simulink model "r2_b16a4x512f"  (R2012b)
settings: Solver=VariableStepDiscrete  SolverMode=SingleTasking  StartTime=0.0  StopTime=1  RelTol=1e-3
undefined symbols (not defined in the file): fft_stages, n_bits_ants, n_bits_xengs
libraries: xbsIndex_r4 x27410, casper_library_misc x230, xbsReplacements_r4 x24, casper_library_delays x8, xps_library x5, casper_library_communications x4
(part 90 of 229)

== system r2_b16a4x512f/sys3/pkt_reord_devel/munge1 ==
  din : Inport
  join : Subsystem  AncestorBlock=casper_library_flow_control/bus_create  mask(bus_create){inputNum=2}
      mask prompts: inputNum "Number of inputs:"
      mask init:
      | bus_create_init(gcb,...
      |     'inputNum', inputNum);
  reinterpret : xbsIndex_r4/Reinterpret  force_arith_type=on  arith_type=Unsigned  force_bin_pt=on  bin_pt=0  block_type=reinterpret
  reinterpret_out : xbsIndex_r4/Reinterpret  force_arith_type=on  arith_type=Unsigned  force_bin_pt=on  bin_pt=0  block_type=reinterpret
  split : Subsystem  AncestorBlock=casper_library_flow_control/bus_expand  mask(bus_expand){mode=divisions of arbitrary size, outputNum=1, outputWidth=[1 32], outputBinaryPt=[0 0], outputArithmeticType=[0 0], show_format=off, outputToWorkspace=off, variablePrefix=out, outputToModelAsWell=on}
      mask prompts: outputNum "Number of outputs:"; outputWidth "Output width [msb ... lsb]:"; outputBinaryPt "Output binary point position [msb ... lsb]:"; outputArithmeticType "Output arithmetic type (ufix=0, fix=1, bool=2) [msb ... lsb]:"; show_format "Print format string?"; outputToWorkspace "Output to workspace?"; variablePrefix "Variable name prefix:"; outputToModelAsWell "Output to model as well?"
      mask help:
      | Expands a 'bus' made using a bus_create or Xilinx
      | concat block.
      | The input will be divided into the specified number
      | of outputs with the specified arithmetic types.
      | Divisions are made from most significant bit.
      mask init: same as r2_b16a4x512f/bus_expand
      settings: AttributesFormatString=2 outputs
      mask TypeOptions mode: divisions of equal size | divisions of arbitrary size
      mask Callback mode: bus_expand_callback();
      mask Callback outputWidth: bus_expand_callback();
      mask Callback outputToWorkspace: bus_expand_callback();
  dout : Outport
  wires:
  split/2(lsb_out1) -> join/2(in2)
  split/1(msb_out2) -> join/1(in1)
  join/1(bus_out) -> reinterpret_out/1
  reinterpret/1 -> split/1(bus_in)
  din/1 -> reinterpret/1
  reinterpret_out/1 -> dout/1

== system r2_b16a4x512f/sys3/pkt_reord_devel/output_control ==
  note: rd_addr is counting for
      | output words to
      | X engines
  note: If the read window is 1/2
      | the total buffer size (or more)
      | behind the write window,
      | it is time to ship it out.
  note: Decide whether to ship
      | a window or not:
  note: If we need to ship a window,
      | send the data on a window edge
  note: If reading from addr 0 (corresponding to f=0,nant,2nant,...)
      | and max_mcnt (skipping window_bits for the difference
      | between max_mcnt and rd_mcnt) is 0 for sync_bits, then
      | issue a sync.
  note: add delay here
      | to ensure mcnt has had
      | chance to calculate
      | correctly
  maxcnt : Inport
  AddSub1 : xbsIndex_r4/AddSub  mode=Subtraction  use_carryin=off  use_carryout=off  en=off  latency=2  precision=User Defined  arith_type=Unsigned  n_bits=window_bits  bin_pt=0  quantization=Truncate  overflow=Wrap  dbl_ovrd=off  use_behavioral_HDL=on  hw_selection=Fabric  pipelined=off  use_rpm=on  block_type=addsub
      settings: xl_area=[0, 0, 0, 0, 0, 0, 0]  block_version=10.1.3
  Concat1 : xbsIndex_r4/Concat  num_inputs=2  dbl_ovrd=off  block_type=concat
      settings: block_version=10.1.3
  Concat2 : xbsIndex_r4/Concat  num_inputs=2  dbl_ovrd=off  block_type=concat
      settings: block_version=10.1.3
  Constant1 : xbsIndex_r4/Constant  const=2^(window_bits - 1)  gui_display_data_type=Fixed-point  arith_type=Unsigned  n_bits=window_bits  bin_pt=0  preci_type=Single  exp_width=8  frac_width=24  explicit_period=on  period=1  equ=P=C  opselect=C  inp2=PCIN>>17  opr=+  inp1=P  carry=CIN  dbl_ovrd=off  block_type=constant
  Constant3 : xbsIndex_r4/Constant  const=0  gui_display_data_type=Fixed-point  arith_type=Unsigned  n_bits=sync_bits - x_int_bits - ant_bits - window_bits  bin_pt=0  preci_type=Single  exp_width=8  frac_width=24  explicit_period=on  period=1  equ=P=C  opselect=C  inp2=PCIN>>17  opr=+  inp1=P  carry=CIN  dbl_ovrd=off  block_type=constant
  Delay1 : xbsIndex_r4/Delay  rst=off  infoeditControl=Selection of Reset will increase slice count due to use of real FFs and instead of SRLs  en=off  latency=1  dbl_ovrd=off  reg_retiming=on  block_type=delay
      settings: xl_area=[0, 0, 0, 0, 0, 0, 0]
  Delay3 : xbsIndex_r4/Delay  rst=off  infoeditControl=Selection of Reset will increase slice count due to use of real FFs and instead of SRLs  en=off  latency=2  dbl_ovrd=off  reg_retiming=on  block_type=delay
      settings: xl_area=[0, 0, 0, 0, 0, 0, 0]
  Delay6 : xbsIndex_r4/Delay  rst=off  infoeditControl=Selection of Reset will increase slice count due to use of real FFs and instead of SRLs  en=off  latency=1  dbl_ovrd=off  reg_retiming=on  block_type=delay
      settings: xl_area=[0, 0, 0, 0, 0, 0, 0]
  Delay7 : xbsIndex_r4/Delay  rst=off  infoeditControl=Selection of Reset will increase slice count due to use of real FFs and instead of SRLs  en=off  latency=2  dbl_ovrd=off  reg_retiming=on  block_type=delay
      settings: xl_area=[0, 0, 0, 0, 0, 0, 0]
  Gateway Out{1..18} (18 alike) : xbsIndex_r4/Gateway Out  inherit_from_input=off  hdl_port=off  timing_constraint=None  locs_specified=off  LOCs={}  UseAsDAC=off  DACChannel='1'  block_type=gatewayout
      settings: infoedit="Gateway out block.  Converts Xilinx fixed point inputs into ouputs of type Simulink integer, double, or fixed point.<P><P>Hardware notes:  In hardware these blocks become top level output ports or are discarded, depending on how they are configured."  xl_area=[0, 0, 0, 0, 0, 0, 0]  block_version=10.1.3
  Logical1 : xbsIndex_r4/Logical  logical_function=AND  inputs=2  en=off  latency=0  precision=Full  arith_type=Unsigned  n_bits=8  bin_pt=2  align_bp=on  dbl_ovrd=off  block_type=logical
      settings: xl_area=[0, 0, 0, 0, 0, 0, 0]
  Logical2 : xbsIndex_r4/Logical  logical_function=AND  inputs=2  en=off  latency=0  precision=Full  arith_type=Unsigned  n_bits=8  bin_pt=2  align_bp=on  dbl_ovrd=off  block_type=logical
      settings: xl_area=[0, 0, 0, 0, 0, 0, 0]
  Logical4 : xbsIndex_r4/Logical  logical_function=AND  inputs=2  en=off  latency=0  precision=Full  arith_type=Unsigned  n_bits=8  bin_pt=2  align_bp=on  dbl_ovrd=off  block_type=logical
      settings: xl_area=[0, 0, 0, 0, 0, 0, 0]
  Register : xbsIndex_r4/Register  init=0  rst=off  en=on  dbl_ovrd=off  block_type=register
  Register1 : xbsIndex_r4/Register  init=0  rst=off  en=on  dbl_ovrd=off  block_type=register
  Register3 : xbsIndex_r4/Register  init=0  rst=off  en=on  dbl_ovrd=off  block_type=register
  Relational1 : xbsIndex_r4/Relational  mode=a>=b  en=off  latency=1  dbl_ovrd=off  block_type=relational
      settings: xl_area=[0, 0, 0, 0, 0, 0, 0]  block_version=10.1.3
  Relational4 : xbsIndex_r4/Relational  mode=a=b  en=off  latency=1  dbl_ovrd=off  block_type=relational
      settings: xl_area=[0, 0, 0, 0, 0, 0, 0]  block_version=10.1.3
  Slice1 : xbsIndex_r4/Slice  nbits=window_bits  boolean_output=off  mode=Lower Bit Location + Width  bit1=0  base1=MSB of Input  bit0=0  base0=LSB of Input  dbl_ovrd=off  block_type=slice
      settings: infoedit="Extracts a given range of bits from each input sample and presents it at the output.  The output type is ordinarily unsigned with binary point at zero, but can be Boolean when the slice is one bit wide.<P><P>Hardware notes: In hardware this block costs nothing."  block_version=10.1.3
  Slice2 : xbsIndex_r4/Slice  nbits=1  boolean_output=on  mode=Upper Bit Location + Width  bit1=0  base1=MSB of Input  bit0=0  base0=LSB of Input  dbl_ovrd=off  block_type=slice
      settings: infoedit="Extracts a given range of bits from each input sample and presents it at the output.  The output type is ordinarily unsigned with binary point at zero, but can be Boolean when the slice is one bit wide.<P><P>Hardware notes: In hardware this block costs nothing."  block_version=10.1.3
  Slice3 : xbsIndex_r4/Slice  nbits=window_bits  boolean_output=off  mode=Lower Bit Location + Width  bit1=0  base1=MSB of Input  bit0=0  base0=LSB of Input  dbl_ovrd=off  block_type=slice
      settings: infoedit="Extracts a given range of bits from each input sample and presents it at the output.  The output type is ordinarily unsigned with binary point at zero, but can be Boolean when the slice is one bit wide.<P><P>Hardware notes: In hardware this block costs nothing."  block_version=10.1.3
  Slice4 : xbsIndex_r4/Slice  nbits=x_int_bits + ant_bits - n_bits_output_words  boolean_output=off  mode=Lower Bit Location + Width  bit1=0  base1=MSB of Input  bit0=0  base0=LSB of Input  dbl_ovrd=off  block_type=slice
      settings: block_version=10.1.3
  Slice5 : xbsIndex_r4/Slice  nbits=window_bits  boolean_output=off  mode=Two Bit Locations  bit1=sync_bits - x_int_bits - ant_bits - 1  base1=LSB of Input  bit0=window_bits  base0=LSB of Input  dbl_ovrd=off  block_type=slice
      settings: infoedit="Extracts a given range of bits from each input sample and presents it at the output.  The output type is ordinarily unsigned with binary point at zero, but can be Boolean when the slice is one bit wide.<P><P>Hardware notes: In hardware this block costs nothing."  block_version=10.1.3
  Slice6 : xbsIndex_r4/Slice  nbits=1  boolean_output=on  mode=Upper Bit Location + Width  bit1=0  base1=MSB of Input  bit0=0  base0=LSB of Input  dbl_ovrd=off  block_type=slice
      settings: infoedit="Extracts a given range of bits from each input sample and presents it at the output.  The output type is ordinarily unsigned with binary point at zero, but can be Boolean when the slice is one bit wide.<P><P>Hardware notes: In hardware this block costs nothing."  block_version=10.1.3
  Slice7 : xbsIndex_r4/Slice  nbits=1  boolean_output=off  mode=Two Bit Locations  bit1=0  base1=MSB of Input  bit0=window_bits  base0=LSB of Input  dbl_ovrd=off  block_type=slice
      settings: infoedit="Extracts a given range of bits from each input sample and presents it at the output.  The output type is ordinarily unsigned with binary point at zero, but can be Boolean when the slice is one bit wide.<P><P>Hardware notes: In hardware this block costs nothing."  block_version=10.1.3
  edge_detect : Subsystem  AncestorBlock=casper_library_misc/edge_detect  mask(edge_detect){edge=Both, polarity=Active High, x_in=[0 0.08 0.08 0.16 0.16 0.24 0.24 0.32 0.32 0.4], y_in=[-1 -1  1  1  1  1  1  1  1  1], x_out=[0.6 0.68 0.68 0.76 0.76 0.84 0.84 0.92 0.92 1], y_out=[-1 -1  1  1 -1 -1 -1 -1 -1 -1]}
      mask prompts: edge "Edge Type"; polarity "Output Polarity"; x_in "Input X Positions"; y_in "Input Y Positions"; x_out "Output X Positions"; y_out "Output Y Positions"
      mask help: Output is active for one-cycle after each edge of the specified type (i.e. rising, falling or both).
      mask init: same as r2_b16a4x512f/edge_detect
      settings: AttributesFormatString=|
      | both edges
      | active high
      mask Help: Output is active for one-cycle after each edge of the specified type (i.e. rising, falling, or both).  Latency is zero.
      mask TypeOptions edge: Rising | Falling | Both
      mask TypeOptions polarity: Active High | Active Low
      mask Display:
      | plot(x_in_num,0.5+y_in_num*0.2);
      | plot(x_out_num,0.5+y_out_num*0.2);
  edge_detect1 : Subsystem  AncestorBlock=casper_library_misc/edge_detect  mask(edge_detect){edge=Both, polarity=Active High, x_in=[0 0.08 0.08 0.16 0.16 0.24 0.24 0.32 0.32 0.4], y_in=[-1 -1  1  1  1  1  1  1  1  1], x_out=[0.6 0.68 0.68 0.76 0.76 0.84 0.84 0.92 0.92 1], y_out=[-1 -1  1  1 -1 -1 -1 -1 -1 -1]}
      mask prompts: edge "Edge Type"; polarity "Output Polarity"; x_in "Input X Positions"; y_in "Input Y Positions"; x_out "Output X Positions"; y_out "Output Y Positions"
      mask help: Output is active for one-cycle after each edge of the specified type (i.e. rising, falling or both).
      mask init: same as r2_b16a4x512f/edge_detect
      settings: AttributesFormatString=|
      | both edges
      | active high
      mask Help: Output is active for one-cycle after each edge of the specified type (i.e. rising, falling, or both).  Latency is zero.
      mask TypeOptions edge: Rising | Falling | Both
      mask TypeOptions polarity: Active High | Active Low
      mask Display:
      | plot(x_in_num,0.5+y_in_num*0.2);
      | plot(x_out_num,0.5+y_out_num*0.2);
  internal_descr_Scope : Scope  NumInputPorts=8
      settings: TimeRange=1  YMin=-1~-1~0.95~-5~-5~-5~-5~-5  YMax=1~1~1.05~5~5~5~5~5  SaveName=ScopeData2
  internal_descr_Scope1 : Scope  NumInputPorts=10
      settings: TimeRange=42.38350921521942  YMin=100.7~0~0~0~402.8~0.95~304~-1~-5~-5  YMax=111.3~10~80~1024~445.2~1.05~336~1~5~5  SaveName=ScopeData4
  pulse_ext : Subsystem  AncestorBlock=casper_library/Misc/pulse_ext  mask(pulse_ext){pulse_len=2^(x_int_bits + ant_bits)}
      mask prompts: pulse_len "Length of Pulse"
      mask help:
      | Extends a boolean signal to be high for the specified number of clocks after
      | the last high input.
      mask init:
      | bits = ceil(log2(pulse_len+1));
      mask Help: eval('xlWeb([getenv(''MLIB_ROOT''), ''\doc\htmlblocks\sp_pulse_ext\sp_pulse_ext.html''])')
  win_addr_cnt : xbsIndex_r4/Counter  cnt_type=Free Running  cnt_to=Inf  operation=Up  start_count=0  cnt_by_val=1  arith_type=Unsigned  n_bits=x_int_bits + ant_bits + 1 - n_bits_output_words  bin_pt=0  load_pin=off  rst=off  en=off  explicit_period=on  period=1  dbl_ovrd=off  use_behavioral_HDL=off  implementation=Fabric  use_rpm=on  block_type=counter
      settings: xl_area=[0, 0, 0, 0, 0, 0, 0]
  win_cnt : xbsIndex_r4/Counter  cnt_type=Free Running  cnt_to=Inf  operation=Up  start_count=0  cnt_by_val=1  arith_type=Unsigned  n_bits=window_bits + 1  bin_pt=0  load_pin=off  rst=off  en=on  explicit_period=off  period=1  dbl_ovrd=off  use_behavioral_HDL=off  implementation=Fabric  use_rpm=on  block_type=counter
      settings: xl_area=[0, 0, 0, 0, 0, 0, 0]
  gen_sync : Outport
  rd_en : Outport  Port=2
  rd_addr : Outport  Port=3
  rd_timefreq : Outport  Port=4
  wires:
  Concat2/1 -> [rd_mcnt], rd_timefreq/1
  Concat1/1 -> rd_addr/1, [rd_addr]
  Delay7/1 -> Concat1/2
  Slice2/1 -> edge_detect/1(in)
  Slice1/1 -> [current_window], Delay1/1
  Slice4/1 -> Delay7/1
  edge_detect1/1(out) -> Logical1/1
  Slice6/1 -> edge_detect1/1(in)
  win_addr_cnt/1 -> Slice4/1, Slice6/1
  Slice5/1 -> Relational4/2
  Constant3/1 -> Relational4/1
  edge_detect/1(out) -> Logical2/1, [buffer_edge]
  Logical1/1 -> Register3/1, Register3/2, pulse_ext/1(in), [ship_window_now]
  Register1/1 -> Slice2/1, Slice1/1
  maxcnt/1 -> Slice5/1, [maxcnt]
  [ship_next_window] -> Delay3/1
  Slice3/1 -> AddSub1/1
  AddSub1/1 -> Relational1/1
  Constant1/1 -> Relational1/2
  [current_window] -> AddSub1/2
  [maxcnt] -> Slice3/1
  Relational1/1 -> [ship_next_window]
  [ship_window_now] -> win_cnt/1, Register1/2
  Relational4/1 -> Logical2/2
  Gateway Out3/1 -> internal_descr_Scope/2
  Gateway Out4/1 -> internal_descr_Scope/1
  Gateway Out5/1 -> internal_descr_Scope/3
  [maxcnt] -> Gateway Out4/1
  [current_window_out] -> Gateway Out3/1
  [ship_next_window] -> Gateway Out5/1
  Gateway Out6/1 -> internal_descr_Scope/4
  Gateway Out1/1 -> internal_descr_Scope/5
  Gateway Out2/1 -> internal_descr_Scope/6
  [ship_window_now] -> Gateway Out6/1
  Gateway Out7/1 -> internal_descr_Scope/7
  [current_window_out] -> Concat2/2
  Gateway Out10/1 -> internal_descr_Scope1/2
  Gateway Out11/1 -> internal_descr_Scope1/1
  Gateway Out12/1 -> internal_descr_Scope1/3
  Gateway Out13/1 -> internal_descr_Scope1/4
  Gateway Out8/1 -> internal_descr_Scope1/5
  Gateway Out9/1 -> internal_descr_Scope1/6
  Gateway Out14/1 -> internal_descr_Scope1/7
  Gateway Out15/1 -> internal_descr_Scope1/8
  [gen_sync] -> Gateway Out15/1
  [gen_sync] -> Gateway Out16/1
  Gateway Out16/1 -> internal_descr_Scope/8
  Logical2/1 -> gen_sync/1, [gen_sync]
  [rd_mcnt] -> Gateway Out7/1
  Logical4/1 -> rd_en/1, [rd_en]
  pulse_ext/1(out) -> Delay6/1
  Register3/1 -> Logical4/2
  Delay6/1 -> Logical4/1
  win_cnt/1 -> Register1/1
  Delay1/1 -> [current_window_out]
  [current_window_out] -> Gateway Out11/1
  [maxcnt] -> Gateway Out10/1
  [offset_mcnt] -> Gateway Out12/1
  [ship_next_window] -> Gateway Out8/1
  [rd_mcnt] -> Gateway Out13/1
  [rd_en] -> Gateway Out9/1
  [rd_addr] -> Gateway Out14/1
  [rd_en] -> Gateway Out1/1
  [rd_addr] -> Gateway Out2/1
  [mcnt_sample] -> Gateway Out17/1
  Gateway Out17/1 -> internal_descr_Scope1/9
  Delay3/1 -> Logical1/2
  [maxcnt] -> Slice7/1, [offset_mcnt]
  Slice7/1 -> Register/1
  Register/1 -> Concat2/1, [sampled_mcnt]
  [sampled_mcnt] -> Gateway Out18/1
  Gateway Out18/1 -> internal_descr_Scope1/10
  [buffer_edge] -> Register/2, [mcnt_sample]
  [current_window_out] -> Concat1/1

== system r2_b16a4x512f/sys3/pkt_reord_devel/time_freq_unpack ==
  din : Inport
  xeng_id : Inport  Port=2
  Concat2 : xbsIndex_r4/Concat  num_inputs=2  dbl_ovrd=off  block_type=concat
  Slice2 : xbsIndex_r4/Slice  nbits=chan_bits-xeng_bits  boolean_output=off  mode=Lower Bit Location + Width  bit1=-1  base1=MSB of Input  bit0=0  base0=LSB of Input  dbl_ovrd=off  block_type=slice
      settings: block_version=10.1.3
  Slice3 : xbsIndex_r4/Slice  nbits=1  boolean_output=off  mode=Two Bit Locations  bit1=0  base1=MSB of Input  bit0=chan_bits-xeng_bits  base0=LSB of Input  dbl_ovrd=off  block_type=slice
      settings: block_version=10.1.3
  time : Outport
  freq : Outport  Port=2
  wires:
  din/1 -> Slice3/1, Slice2/1
  Slice3/1 -> time/1
  Slice2/1 -> Concat2/2
  Concat2/1 -> freq/1
  xeng_id/1 -> Concat2/1

== system r2_b16a4x512f/sys3/pre_process/bus_expand ==
  bus_in : Inport
  reinterpret{1..4} (4 alike) : xbsIndex_r4/Reinterpret  force_arith_type=on  arith_type=Unsigned  force_bin_pt=on  bin_pt=0  block_type=reinterpret
  slice1 : xbsIndex_r4/Slice  nbits=8  boolean_output=off  mode=Upper Bit Location + Width  bit1=-40  base1=MSB of Input  bit0=0  base0=LSB of Input  dbl_ovrd=off  block_type=slice
  slice2 : xbsIndex_r4/Slice  nbits=16  boolean_output=off  mode=Upper Bit Location + Width  bit1=-24  base1=MSB of Input  bit0=0  base0=LSB of Input  dbl_ovrd=off  block_type=slice
  slice3 : xbsIndex_r4/Slice  nbits=8  boolean_output=off  mode=Upper Bit Location + Width  bit1=-16  base1=MSB of Input  bit0=0  base0=LSB of Input  dbl_ovrd=off  block_type=slice
  slice4 : xbsIndex_r4/Slice  nbits=16  boolean_output=off  mode=Upper Bit Location + Width  bit1=0  base1=MSB of Input  bit0=0  base0=LSB of Input  dbl_ovrd=off  block_type=slice
  msb_out4 : Outport
  out3 : Outport  Port=2
  out2 : Outport  Port=3
  lsb_out1 : Outport  Port=4
  wires:
  bus_in/1 -> slice4/1, slice3/1, slice2/1, slice1/1
  slice4/1 -> reinterpret4/1
  reinterpret4/1 -> msb_out4/1
  slice3/1 -> reinterpret3/1
  reinterpret3/1 -> out3/1
  slice2/1 -> reinterpret2/1
  reinterpret2/1 -> out2/1
  slice1/1 -> reinterpret1/1
  reinterpret1/1 -> lsb_out1/1

== system r2_b16a4x512f/sys3/pre_process/bus_expand1 ==
  bus_in : Inport
  reinterpret{1..5} (5 alike) : xbsIndex_r4/Reinterpret  force_arith_type=on  arith_type=Unsigned  force_bin_pt=on  bin_pt=0  block_type=reinterpret
  slice1 : xbsIndex_r4/Slice  nbits=1  boolean_output=off  mode=Upper Bit Location + Width  bit1=-7  base1=MSB of Input  bit0=0  base0=LSB of Input  dbl_ovrd=off  block_type=slice
  slice2 : xbsIndex_r4/Slice  nbits=1  boolean_output=off  mode=Upper Bit Location + Width  bit1=-6  base1=MSB of Input  bit0=0  base0=LSB of Input  dbl_ovrd=off  block_type=slice
  slice3 : xbsIndex_r4/Slice  nbits=1  boolean_output=off  mode=Upper Bit Location + Width  bit1=-5  base1=MSB of Input  bit0=0  base0=LSB of Input  dbl_ovrd=off  block_type=slice
  slice4 : xbsIndex_r4/Slice  nbits=1  boolean_output=off  mode=Upper Bit Location + Width  bit1=-4  base1=MSB of Input  bit0=0  base0=LSB of Input  dbl_ovrd=off  block_type=slice
  slice5 : xbsIndex_r4/Slice  nbits=4  boolean_output=off  mode=Upper Bit Location + Width  bit1=0  base1=MSB of Input  bit0=0  base0=LSB of Input  dbl_ovrd=off  block_type=slice
  msb_out5 : Outport
  out4 : Outport  Port=2
  out3 : Outport  Port=3
  out2 : Outport  Port=4
  lsb_out1 : Outport  Port=5
  wires:
  bus_in/1 -> slice5/1, slice4/1, slice3/1, slice2/1, slice1/1
  slice5/1 -> reinterpret5/1
  reinterpret5/1 -> msb_out5/1
  slice4/1 -> reinterpret4/1
  reinterpret4/1 -> out4/1
  slice3/1 -> reinterpret3/1
  reinterpret3/1 -> out3/1
  slice2/1 -> reinterpret2/1
  reinterpret2/1 -> out2/1
  slice1/1 -> reinterpret1/1
  reinterpret1/1 -> lsb_out1/1

== system r2_b16a4x512f/sys3/pre_process/bus_expand2 ==
  bus_in : Inport
  reinterpret{1..12} (12 alike) : xbsIndex_r4/Reinterpret  force_arith_type=on  arith_type=Unsigned  force_bin_pt=on  bin_pt=0  block_type=reinterpret
  slice1 : xbsIndex_r4/Slice  nbits=1  boolean_output=off  mode=Upper Bit Location + Width  bit1=-15  base1=MSB of Input  bit0=0  base0=LSB of Input  dbl_ovrd=off  block_type=slice
  slice10 : xbsIndex_r4/Slice  nbits=1  boolean_output=off  mode=Upper Bit Location + Width  bit1=-6  base1=MSB of Input  bit0=0  base0=LSB of Input  dbl_ovrd=off  block_type=slice
  slice11 : xbsIndex_r4/Slice  nbits=1  boolean_output=off  mode=Upper Bit Location + Width  bit1=-5  base1=MSB of Input  bit0=0  base0=LSB of Input  dbl_ovrd=off  block_type=slice
  slice12 : xbsIndex_r4/Slice  nbits=5  boolean_output=off  mode=Upper Bit Location + Width  bit1=0  base1=MSB of Input  bit0=0  base0=LSB of Input  dbl_ovrd=off  block_type=slice
  slice2 : xbsIndex_r4/Slice  nbits=1  boolean_output=off  mode=Upper Bit Location + Width  bit1=-14  base1=MSB of Input  bit0=0  base0=LSB of Input  dbl_ovrd=off  block_type=slice
  slice3 : xbsIndex_r4/Slice  nbits=1  boolean_output=off  mode=Upper Bit Location + Width  bit1=-13  base1=MSB of Input  bit0=0  base0=LSB of Input  dbl_ovrd=off  block_type=slice
  slice4 : xbsIndex_r4/Slice  nbits=1  boolean_output=off  mode=Upper Bit Location + Width  bit1=-12  base1=MSB of Input  bit0=0  base0=LSB of Input  dbl_ovrd=off  block_type=slice
  slice5 : xbsIndex_r4/Slice  nbits=1  boolean_output=off  mode=Upper Bit Location + Width  bit1=-11  base1=MSB of Input  bit0=0  base0=LSB of Input  dbl_ovrd=off  block_type=slice
  slice6 : xbsIndex_r4/Slice  nbits=1  boolean_output=off  mode=Upper Bit Location + Width  bit1=-10  base1=MSB of Input  bit0=0  base0=LSB of Input  dbl_ovrd=off  block_type=slice
  slice7 : xbsIndex_r4/Slice  nbits=1  boolean_output=off  mode=Upper Bit Location + Width  bit1=-9  base1=MSB of Input  bit0=0  base0=LSB of Input  dbl_ovrd=off  block_type=slice
  slice8 : xbsIndex_r4/Slice  nbits=1  boolean_output=off  mode=Upper Bit Location + Width  bit1=-8  base1=MSB of Input  bit0=0  base0=LSB of Input  dbl_ovrd=off  block_type=slice
  slice9 : xbsIndex_r4/Slice  nbits=1  boolean_output=off  mode=Upper Bit Location + Width  bit1=-7  base1=MSB of Input  bit0=0  base0=LSB of Input  dbl_ovrd=off  block_type=slice
  msb_out12 : Outport
  out11 : Outport  Port=2
  out10 : Outport  Port=3
  out9 : Outport  Port=4
  out8 : Outport  Port=5
  out7 : Outport  Port=6
  out6 : Outport  Port=7
  out5 : Outport  Port=8
  out4 : Outport  Port=9
  out3 : Outport  Port=10
  out2 : Outport  Port=11
  lsb_out1 : Outport  Port=12
  wires:
  bus_in/1 -> slice12/1, slice11/1, slice10/1, slice9/1, slice8/1, slice7/1, slice6/1, slice5/1, slice4/1, slice3/1, slice2/1, slice1/1
  slice12/1 -> reinterpret12/1
  reinterpret12/1 -> msb_out12/1
  slice11/1 -> reinterpret11/1
  reinterpret11/1 -> out11/1
  slice10/1 -> reinterpret10/1
  reinterpret10/1 -> out10/1
  slice9/1 -> reinterpret9/1
  reinterpret9/1 -> out9/1
  slice8/1 -> reinterpret8/1
  reinterpret8/1 -> out8/1
  slice7/1 -> reinterpret7/1
  reinterpret7/1 -> out7/1
  slice6/1 -> reinterpret6/1
  reinterpret6/1 -> out6/1
  slice5/1 -> reinterpret5/1
  reinterpret5/1 -> out5/1
  slice4/1 -> reinterpret4/1
  reinterpret4/1 -> out4/1
  slice3/1 -> reinterpret3/1
  reinterpret3/1 -> out3/1
  slice2/1 -> reinterpret2/1
  reinterpret2/1 -> out2/1
  slice1/1 -> reinterpret1/1
  reinterpret1/1 -> lsb_out1/1

== system r2_b16a4x512f/sys3/speadify0/data_fifo ==
  note: reverse word
      | order on way out
  note: top two bits both going
      | low indicates roll over
      | from max to 0 i.e overflow
  rst : Inport
  we : Inport  Port=2
  di : Inport  Port=3
  re : Inport  Port=4
  %full_calc : xbsIndex_r4/AddSub  mode=Subtraction  use_carryin=off  use_carryout=off  en=off  latency=1  precision=User Defined  arith_type=Unsigned  n_bits=depth_bits-scale_bits  bin_pt=0  quantization=Truncate  overflow=Wrap  dbl_ovrd=off  use_behavioral_HDL=off  hw_selection=Fabric  pipelined=off  block_type=addsub
  %full_slc : xbsIndex_r4/Slice  nbits=full_bits  boolean_output=off  mode=Upper Bit Location + Width  bit1=0  base1=MSB of Input  bit0=0  base0=LSB of Input  dbl_ovrd=off  block_type=slice
  Constant : xbsIndex_r4/Constant  const=0  gui_display_data_type=Fixed-point  arith_type=Boolean  n_bits=16  bin_pt=14  preci_type=Single  exp_width=8  frac_width=24  explicit_period=off  period=1  equ=P=C  opselect=C  inp2=PCIN>>17  opr=+  inp1=P  carry=CIN  dbl_ovrd=off  block_type=constant
      settings: block_version=11.4
  Gateway Out{,1..4} (5 alike) : xbsIndex_r4/Gateway Out  inherit_from_input=off  hdl_port=off  timing_constraint=None  locs_specified=off  LOCs={}  UseAsDAC=off  DACChannel='1'  block_type=gatewayout
      settings: infoedit="Gateway out block.  Converts Xilinx fixed point inputs into ouputs of type Simulink integer, double, or fixed point.<br><br>Hardware notes:  In hardware these blocks become top level output ports or are discarded, depending on how they are configured."  block_version=11.4
  Logical : xbsIndex_r4/Logical  logical_function=AND  inputs=2  en=off  latency=0  precision=Full  arith_type=Unsigned  n_bits=16  bin_pt=0  align_bp=on  dbl_ovrd=off  block_type=logical
      settings: block_version=11.4
  Scope : Scope  NumInputPorts=5
      settings: YMin=0~0~0~0~-5  YMax=1750~2500~2500~1~5  SaveName=ScopeData13
  Slice1 : xbsIndex_r4/Slice  nbits=depth_bits-scale_bits  boolean_output=off  mode=Upper Bit Location + Width  bit1=0  base1=MSB of Input  bit0=0  base0=LSB of Input  dbl_ovrd=off  block_type=slice
  buf : xbsIndex_r4/Dual Port RAM  depth=2^depth_bits  initVector=zeros(1,2^depth_bits)  distributed_mem=Block RAM  init_a=0  init_b=0  rst_a=off  rst_b=off  en_a=off  en_b=off  latency=1  write_mode_A=Read Before Write  write_mode_B=Read Before Write  dbl_ovrd=off  optimize=Speed  block_type=dpram
      settings: block_version=11.4
  bus_replicate : Subsystem  AncestorBlock=casper_library_bus/bus_replicate  mask(bus_replicate){replication=2^scale_bits, latency=0, misc=off, implementation=core}
      mask prompts: replication "replication factor"; misc "misc support"; implementation "delay implementation"
      mask help: Output bus formed by replicating input bus a number of times
      mask init:
      | bus_replicate_init(gcb, ...
      |     'replication', replication, ...
      |     'latency', latency, ...
      |     'implementation', implementation, ...
      |     'misc', misc);
      mask TypeOptions implementation: core | behavioral
  edge_detect : Subsystem  AncestorBlock=casper_library_misc/edge_detect  mask(edge_detect){edge=Falling, polarity=Active High, x_in=[0 0.08 0.08 0.16 0.16 0.24 0.24 0.32 0.32 0.4], y_in=[1  1 -1 -1 -1 -1 -1 -1 -1 -1], x_out=[0.6 0.68 0.68 0.76 0.76 0.84 0.84 0.92 0.92 1], y_out=[-1 -1  1  1 -1 -1 -1 -1 -1 -1]}
      mask prompts: edge "Edge Type"; polarity "Output Polarity"; x_in "Input X Positions"; y_in "Input Y Positions"; x_out "Output X Positions"; y_out "Output Y Positions"
      mask help: Output is active for one-cycle after each edge of the specified type (i.e. rising, falling or both).
      mask init: same as r2_b16a4x512f/edge_detect
      settings: AttributesFormatString=|
      | falling edges
      | active high
      mask Help: Output is active for one-cycle after each edge of the specified type (i.e. rising, falling, or both).  Latency is zero.
      mask TypeOptions edge: Rising | Falling | Both
      mask TypeOptions polarity: Active High | Active Low
      mask Display:
      | plot(x_in_num,0.5+y_in_num*0.2);
      | plot(x_out_num,0.5+y_out_num*0.2);
  edge_detect1 : Subsystem  AncestorBlock=casper_library_misc/edge_detect  mask(edge_detect){edge=Falling, polarity=Active High, x_in=[0 0.08 0.08 0.16 0.16 0.24 0.24 0.32 0.32 0.4], y_in=[1  1 -1 -1 -1 -1 -1 -1 -1 -1], x_out=[0.6 0.68 0.68 0.76 0.76 0.84 0.84 0.92 0.92 1], y_out=[-1 -1  1  1 -1 -1 -1 -1 -1 -1]}
      mask prompts: edge "Edge Type"; polarity "Output Polarity"; x_in "Input X Positions"; y_in "Input Y Positions"; x_out "Output X Positions"; y_out "Output Y Positions"
      mask help: Output is active for one-cycle after each edge of the specified type (i.e. rising, falling or both).
      mask init: same as r2_b16a4x512f/edge_detect
      settings: AttributesFormatString=|
      | falling edges
      | active high
      mask Help: Output is active for one-cycle after each edge of the specified type (i.e. rising, falling, or both).  Latency is zero.
      mask TypeOptions edge: Rising | Falling | Both
      mask TypeOptions polarity: Active High | Active Low
      mask Display:
      | plot(x_in_num,0.5+y_in_num*0.2);
      | plot(x_out_num,0.5+y_out_num*0.2);
  msb : xbsIndex_r4/Slice  nbits=1  boolean_output=on  mode=Upper Bit Location + Width  bit1=0  base1=MSB of Input  bit0=0  base0=LSB of Input  dbl_ovrd=off  block_type=slice
  msb-1 : xbsIndex_r4/Slice  nbits=1  boolean_output=on  mode=Upper Bit Location + Width  bit1=-1  base1=MSB of Input  bit0=0  base0=LSB of Input  dbl_ovrd=off  block_type=slice
  munge : Subsystem  AncestorBlock=casper_library_flow_control/munge  mask(munge){divisions=2^scale_bits, div_size=repmat(n_bits_in, 1, 2^scale_bits), order=[2^scale_bits-1:-1:0]}
      mask prompts: divisions "Number of divisions"; div_size "Division size (bits)"; order "Division packing order"
      mask help: Splits an input bus into the specified number of divisions and then recombines them in the order specified (most significant division = 0,least = number divisions-1)
      mask init:
      | munge_init(gcb, ...
      |     'divisions', divisions, ...
      |     'div_size', div_size, ...
      |     'order', order);
      settings: AttributesFormatString=|
      | split:[16 16 16 16]
      | join:[3 2 1 0]
      | Unsigned [64,0]
  rd_add : xbsIndex_r4/Counter  cnt_type=Free Running  cnt_to=Inf  operation=Up  start_count=0  cnt_by_val=1  arith_type=Unsigned  n_bits=depth_bits-scale_bits  bin_pt=0  load_pin=off  rst=on  en=on  explicit_period=on  period=1  dbl_ovrd=off  use_behavioral_HDL=on  implementation=Fabric  block_type=counter
      settings: block_version=11.4
  wr_add : xbsIndex_r4/Counter  cnt_type=Free Running  cnt_to=Inf  operation=Up  start_count=0  cnt_by_val=1  arith_type=Unsigned  n_bits=depth_bits  bin_pt=0  load_pin=off  rst=on  en=on  explicit_period=on  period=1  dbl_ovrd=off  use_behavioral_HDL=on  implementation=Fabric  block_type=counter
      settings: block_version=11.4
  do : Outport
  %full : Outport  Port=2
  of : Outport  Port=3
  wires:
  wr_add/1 -> buf/1, Slice1/1, Gateway Out/1
  we/1 -> wr_add/2, buf/3
  rd_add/1 -> buf/4, %full_calc/2, Gateway Out1/1
  rst/1 -> rd_add/1, wr_add/1
  %full_calc/1 -> Gateway Out2/1, %full_slc/1, msb/1, msb-1/1
  di/1 -> buf/2
  re/1 -> rd_add/2
  buf/2 -> munge/1(din)
  Slice1/1 -> %full_calc/1
  %full_slc/1 -> %full/1, Gateway Out3/1
  Constant/1 -> buf/6
  bus_replicate/1(out) -> buf/5
  buf/1 -> bus_replicate/1(in)
  Gateway Out/1 -> Scope/1
  Gateway Out1/1 -> Scope/2
  Gateway Out2/1 -> Scope/3
  Gateway Out3/1 -> Scope/4
  munge/1(dout) -> do/1
  msb/1 -> edge_detect/1(in)
  msb-1/1 -> edge_detect1/1(in)
  edge_detect/1(out) -> Logical/1
  edge_detect1/1(out) -> Logical/2
  Logical/1 -> of/1, Gateway Out4/1
  Gateway Out4/1 -> Scope/5

== system r2_b16a4x512f/sys3/speadify0/edge_detect ==
  in : Inport
  Delay : xbsIndex_r4/Delay  rst=off  infoeditControl=Selection of Reset will increase slice count due to use of real FFs and instead of SRLs  en=off  latency=1  dbl_ovrd=off  reg_retiming=on  block_type=delay
      settings: xl_area=[0, 0, 0, 0, 0, 0, 0]
  Inverter : xbsIndex_r4/Inverter  en=off  latency=0  dbl_ovrd=off  block_type=inv
      settings: xl_area=[0, 0, 0, 0, 0, 0, 0]
  edge_op : xbsIndex_r4/Logical  logical_function=NOR  inputs=2  en=off  latency=0  precision=Full  arith_type=Unsigned  n_bits=8  bin_pt=2  align_bp=on  dbl_ovrd=off  block_type=logical
      settings: xl_area=[0, 0, 0, 0, 0, 0, 0]
  out : Outport
  wires:
  Inverter/1 -> edge_op/1
  edge_op/1 -> out/1
  in/1 -> Inverter/1, Delay/1
  Delay/1 -> edge_op/2

== system r2_b16a4x512f/sys3/speadify0/edge_detect2 ==
  in : Inport
  Delay : xbsIndex_r4/Delay  rst=off  infoeditControl=Selection of Reset will increase slice count due to use of real FFs and instead of SRLs  en=off  latency=1  dbl_ovrd=off  reg_retiming=on  block_type=delay
      settings: xl_area=[0, 0, 0, 0, 0, 0, 0]
  Inverter : xbsIndex_r4/Inverter  en=off  latency=0  dbl_ovrd=off  block_type=inv
      settings: xl_area=[0, 0, 0, 0, 0, 0, 0]
  edge_op : xbsIndex_r4/Logical  logical_function=NOR  inputs=2  en=off  latency=0  precision=Full  arith_type=Unsigned  n_bits=8  bin_pt=2  align_bp=on  dbl_ovrd=off  block_type=logical
      settings: xl_area=[0, 0, 0, 0, 0, 0, 0]
  out : Outport
  wires:
  Inverter/1 -> edge_op/1
  edge_op/1 -> out/1
  in/1 -> Inverter/1, Delay/1
  Delay/1 -> edge_op/2

== system r2_b16a4x512f/sys3/speadify0/edge_detect3 ==
  in : Inport
  Delay : xbsIndex_r4/Delay  rst=off  infoeditControl=Selection of Reset will increase slice count due to use of real FFs and instead of SRLs  en=off  latency=1  dbl_ovrd=off  reg_retiming=on  block_type=delay
      settings: xl_area=[0, 0, 0, 0, 0, 0, 0]
  Inverter : xbsIndex_r4/Inverter  en=off  latency=0  dbl_ovrd=off  block_type=inv
      settings: xl_area=[0, 0, 0, 0, 0, 0, 0]
  edge_op : xbsIndex_r4/Logical  logical_function=NOR  inputs=2  en=off  latency=0  precision=Full  arith_type=Unsigned  n_bits=8  bin_pt=2  align_bp=on  dbl_ovrd=off  block_type=logical
      settings: xl_area=[0, 0, 0, 0, 0, 0, 0]
  out : Outport
  wires:
  Inverter/1 -> edge_op/1
  edge_op/1 -> out/1
  in/1 -> Inverter/1, Delay/1
  Delay/1 -> edge_op/2

== system r2_b16a4x512f/sys3/speadify0/edge_detect4 ==
  in : Inport
  Delay : xbsIndex_r4/Delay  rst=off  infoeditControl=Selection of Reset will increase slice count due to use of real FFs and instead of SRLs  en=off  latency=1  dbl_ovrd=off  reg_retiming=on  block_type=delay
      settings: xl_area=[0, 0, 0, 0, 0, 0, 0]
  Inverter : xbsIndex_r4/Inverter  en=off  latency=0  dbl_ovrd=off  block_type=inv
      settings: xl_area=[0, 0, 0, 0, 0, 0, 0]
  edge_op : xbsIndex_r4/Logical  logical_function=NOR  inputs=2  en=off  latency=0  precision=Full  arith_type=Unsigned  n_bits=8  bin_pt=2  align_bp=on  dbl_ovrd=off  block_type=logical
      settings: xl_area=[0, 0, 0, 0, 0, 0, 0]
  out : Outport
  wires:
  Delay/1 -> edge_op/2
  in/1 -> Delay/1, Inverter/1
  edge_op/1 -> out/1
  Inverter/1 -> edge_op/1

== system r2_b16a4x512f/sys3/speadify0/edge_detect7 ==
  in : Inport
  Delay : xbsIndex_r4/Delay  rst=off  infoeditControl=Selection of Reset will increase slice count due to use of real FFs and instead of SRLs  en=off  latency=1  dbl_ovrd=off  reg_retiming=on  block_type=delay
      settings: xl_area=[0, 0, 0, 0, 0, 0, 0]
  Inverter : xbsIndex_r4/Inverter  en=off  latency=0  dbl_ovrd=off  block_type=inv
      settings: xl_area=[0, 0, 0, 0, 0, 0, 0]
  edge_op : xbsIndex_r4/Logical  logical_function=NOR  inputs=2  en=off  latency=0  precision=Full  arith_type=Unsigned  n_bits=8  bin_pt=2  align_bp=on  dbl_ovrd=off  block_type=logical
      settings: xl_area=[0, 0, 0, 0, 0, 0, 0]
  out : Outport
  wires:
  Inverter/1 -> edge_op/1
  edge_op/1 -> out/1
  in/1 -> Inverter/1, Delay/1
  Delay/1 -> edge_op/2

== system r2_b16a4x512f/sys3/speadify0/pack ==
  pkt_rdy : Inport
  Assert5 : xbsIndex_r4/Assert  assert_type=on  type_source=Explicitly  gui_display_data_type=Fixed-point  arith_type=Boolean  n_bits=64  bin_pt=0  preci_type=Single  exp_width=8  frac_width=24  assert_rate=off  rate_source=Explicitly  period=1  output_port=on  block_type=assert
      settings: block_version=10.1.3
  Constant2 : xbsIndex_r4/Constant  const=(2^(pkt_bits))-1  gui_display_data_type=Fixed-point  arith_type=Unsigned  n_bits=pkt_bits+1  bin_pt=0  preci_type=Single  exp_width=8  frac_width=24  explicit_period=on  period=1  equ=P=C  opselect=C  inp2=PCIN>>17  opr=+  inp1=P  carry=CIN  dbl_ovrd=off  block_type=constant
  Counter1 : xbsIndex_r4/Counter  cnt_type=Free Running  cnt_to=1023  operation=Up  start_count=0  cnt_by_val=1  arith_type=Unsigned  n_bits=pkt_bits+1  bin_pt=0  load_pin=off  rst=on  en=on  explicit_period=on  period=1  dbl_ovrd=off  use_behavioral_HDL=off  implementation=Fabric  use_rpm=on  block_type=counter
      settings: xl_area=[0, 0, 0, 0, 0, 0, 0]
  Inverter1 : xbsIndex_r4/Inverter  en=off  latency=0  dbl_ovrd=off  block_type=inv
      settings: xl_area=[0, 0, 0, 0, 0, 0, 0]
  Logical2 : xbsIndex_r4/Logical  logical_function=AND  inputs=2  en=off  latency=0  precision=Full  arith_type=Unsigned  n_bits=8  bin_pt=2  align_bp=on  dbl_ovrd=off  block_type=logical
      settings: xl_area=[0, 0, 0, 0, 0, 0, 0]
  Logical4 : xbsIndex_r4/Logical  logical_function=AND  inputs=2  en=off  latency=0  precision=Full  arith_type=Unsigned  n_bits=8  bin_pt=2  align_bp=on  dbl_ovrd=off  block_type=logical
      settings: xl_area=[0, 0, 0, 0, 0, 0, 0]
  Register : xbsIndex_r4/Register  init=0  rst=on  en=on  dbl_ovrd=off  block_type=register
      settings: block_version=11.4
  Relational3 : xbsIndex_r4/Relational  mode=a<=b  en=off  latency=0  dbl_ovrd=off  block_type=relational
      settings: xl_area=[0, 0, 0, 0, 0, 0, 0]  block_version=10.1.3
  edge_detect1 : Subsystem  AncestorBlock=casper_library_misc/edge_detect  mask(edge_detect){edge=Falling, polarity=Active High, x_in=[0 0.08 0.08 0.16 0.16 0.24 0.24 0.32 0.32 0.4], y_in=[1  1 -1 -1 -1 -1 -1 -1 -1 -1], x_out=[0.6 0.68 0.68 0.76 0.76 0.84 0.84 0.92 0.92 1], y_out=[-1 -1  1  1 -1 -1 -1 -1 -1 -1]}
      mask prompts: edge "Edge Type"; polarity "Output Polarity"; x_in "Input X Positions"; y_in "Input Y Positions"; x_out "Output X Positions"; y_out "Output Y Positions"
      mask help: Output is active for one-cycle after each edge of the specified type (i.e. rising, falling or both).
      mask init: same as r2_b16a4x512f/edge_detect
      settings: AttributesFormatString=|
      | falling edges
      | active high
      mask Help: Output is active for one-cycle after each edge of the specified type (i.e. rising, falling, or both).  Latency is zero.
      mask TypeOptions edge: Rising | Falling | Both
      mask TypeOptions polarity: Active High | Active Low
      mask Display:
      | plot(x_in_num,0.5+y_in_num*0.2);
      | plot(x_out_num,0.5+y_out_num*0.2);
  edge_detect3 : Subsystem  AncestorBlock=casper_library_misc/edge_detect  mask(edge_detect){edge=Rising, polarity=Active High, x_in=[0 0.08 0.08 0.16 0.16 0.24 0.24 0.32 0.32 0.4], y_in=[-1 -1  1  1  1  1  1  1  1  1], x_out=[0.6 0.68 0.68 0.76 0.76 0.84 0.84 0.92 0.92 1], y_out=[-1 -1  1  1 -1 -1 -1 -1 -1 -1]}
      mask prompts: edge "Edge Type"; polarity "Output Polarity"; x_in "Input X Positions"; y_in "Input Y Positions"; x_out "Output X Positions"; y_out "Output Y Positions"
      mask help: Output is active for one-cycle after each edge of the specified type (i.e. rising, falling or both).
      mask init: same as r2_b16a4x512f/edge_detect
      settings: AttributesFormatString=|
      | rising edges
      | active high
      mask Help: Output is active for one-cycle after each edge of the specified type (i.e. rising, falling, or both).  Latency is zero.
      mask TypeOptions edge: Rising | Falling | Both
      mask TypeOptions polarity: Active High | Active Low
      mask Display:
      | plot(x_in_num,0.5+y_in_num*0.2);
      | plot(x_out_num,0.5+y_out_num*0.2);
  pkt_start : Outport
  ack_out : Outport  Port=2
  wires:
  [pkt_start] -> Counter1/1
  Assert5/1 -> [pkt_rdy_in]
  pkt_rdy/1 -> Assert5/1
  Counter1/1 -> Relational3/1, [pld_pos]
  Constant2/1 -> Relational3/2
  Relational3/1 -> [writing_pld]
  Logical2/1 -> edge_detect3/1(in)
  [writing_pld] -> Counter1/2
  [pkt_rdy_in] -> Logical2/2
  [pkt_start] -> Register/1, Register/3
  Register/1 -> [busy]
  [busy] -> Inverter1/1
  Inverter1/1 -> Logical2/1
  [writing_pld] -> edge_detect1/1(in)
  edge_detect1/1(out) -> Register/2
  edge_detect3/1(out) -> [pkt_start]
  [rd_data] -> ack_out/1
  [writing_pld] -> Logical4/1
  [busy] -> Logical4/2
  Logical4/1 -> [rd_data]
  [pkt_start] -> pkt_start/1
